simulink model "fullWaveUncontrolledRectifier_Rload"  (R2024b)
settings: Solver=ode23t  StartTime=0.0  StopTime=0.16  MaxStep=1e-4  RelTol=1e-3
libraries: spsDiodeLib x4, spsSeriesRLCBranchLib x3, spsVoltageMeasurementLib x2, spsACVoltageSourceLib x1, spsLinearTransformerLib x1, spsCurrentMeasurementLib x1, sps_lib x1
settings Model: Creator=farha  LastModifiedBy=farha

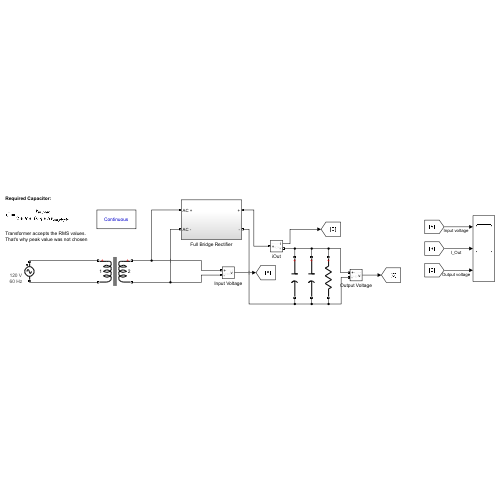
[thumbnail: Simulink's stored preview of the top-level diagram]
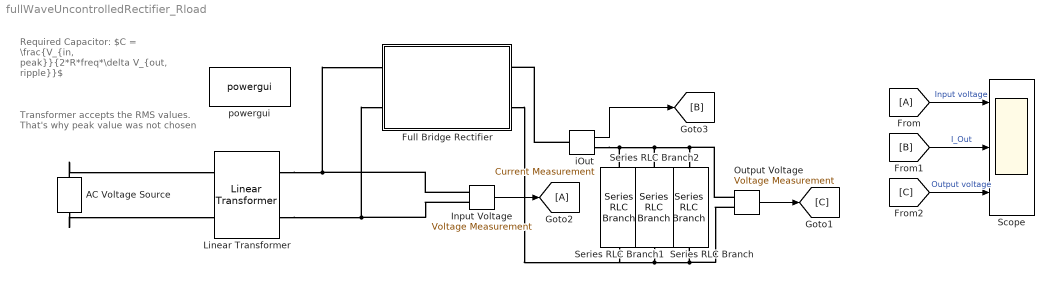
== system fullWaveUncontrolledRectifier_Rload ==
  note: Transformer accepts the RMS values.
      | That's why peak value was not chosen
  note: Required Capacitor:
      |
      | $C = \frac{V_{in, peak}}{2*R*freq*\delta V_{out, ripple}}$
  AC Voltage Source : spsACVoltageSourceLib/AC Voltage Source  Amplitude=120  Phase=0  Frequency=60  SampleTime=0  Measurements=None  BusType=swing  Pref=10e3  Qref=0  Qmin=-inf  Qmax=+inf
      settings: AttributesFormatString=|
      | %<Amplitude> V
      | %<Frequency> Hz
  From : From
  Full Bridge Rectifier : Subsystem
  Goto2 : Goto
  Input Voltage : spsVoltageMeasurementLib/Voltage Measurement  PhasorSimulation=off  OutputType=Complex  PSBequivalent=0
  Linear Transformer : spsLinearTransformerLib/Linear Transformer  UNITS=pu  NominalPower=[ 300 60 ]  winding1=[ 120 0 0 ]  winding2="[ 25.6  0  0 ]"  ThreeWindings=off  winding3=[ 315e3 0.002 0.08 ]  RmLm=[ 500 500 ]  Measurements=None  DataType=off
  Output Voltage : spsVoltageMeasurementLib/Voltage Measurement  PhasorSimulation=off  OutputType=Complex  PSBequivalent=0
  Scope : Scope  NumInputPorts=3
  Series RLC Branch : spsSeriesRLCBranchLib/Series RLC Branch  LConnTagsString=__new0  RConnTagsString=__new0  BranchType=R  Resistance=500  Inductance=1e-3  SetiL0=off  InitialCurrent=0  Capacitance=1e-6  Setx0=off  InitialVoltage=0  Measurements=None
  Series RLC Branch1 : spsSeriesRLCBranchLib/Series RLC Branch  LConnTagsString=__new0  RConnTagsString=__new0  BranchType=C  Resistance=5  Inductance=1e-3  SetiL0=off  InitialCurrent=0  Capacitance=47e-6  Setx0=off  InitialVoltage=0  Measurements=None
  Series RLC Branch2 : spsSeriesRLCBranchLib/Series RLC Branch  LConnTagsString=__new0  RConnTagsString=__new0  BranchType=C  Resistance=5  Inductance=1e-3  SetiL0=off  InitialCurrent=0  Capacitance=47e-6  Setx0=off  InitialVoltage=0  Measurements=None
  iOut : spsCurrentMeasurementLib/Current Measurement  PhasorSimulation=off  OutputType=Complex  PSBequivalent=0
  powergui : sps_lib/powergui  Priority=1  SimulationMode=Continuous  SampleTime=50e-6  frequency=60  Iterations=50  frequencyindice=60  Pbase=100e6  ErrMax=1e-4  UnitsV=kV  UnitsW=MW  buscounter=0  FunctionMessages=off  echomessages=off  EnableUseOfTLC=off  CurrentSourceSwitches=off  DisableSnubberDevices=off  DisableRonSwitches=off  DisableVfSwitches=off  DisplayEquations=off  AutomaticDiscreteSolvers=off  SolverType=Tustin/Backward Euler (TBE)  Interpol=off  ExternalGateDelay=off  methode=off  Ts=100  x0status=blocks  SPID=on  SwTol=0  HookPort=off  NonlinearTolerance=1e-4  nMaxIteration=100  ContinueOnMaxIteration=off  RestoreLinks=warning  ResistiveCurrentMeasurement=off  Frange=[0:2:500]  Ylog=off  Xlog=on  ShowGrid=off  save=off  variable=ZData  structure=0  ZoomFFT=off  StartTime=0.0  cycles=1  DisplayStyle=1  fundamental=60  FreqAxis=off  MaxFrequency=1000  frequencyindicesteady=1  RmsSteady=1  display=off
  wires:
  From/1 -> Scope/1  "Input voltage"
  [B] -> Scope/2  "I_Out"
  [C] -> Scope/3  "Output voltage"
  Output Voltage/1 -> [C]
  iOut/1 -> [B]
  Input Voltage/1 -> Goto2/1
  connections:
  iOut/RConn1 -- Series RLC Branch2/LConn1 -- Output Voltage/LConn1 -- Series RLC Branch/LConn1 -- Series RLC Branch1/LConn1
  Input Voltage/LConn1 -- Full Bridge Rectifier/LConn1 -- Linear Transformer/RConn1
  Input Voltage/LConn2 -- Linear Transformer/RConn2 -- Full Bridge Rectifier/LConn2
  Output Voltage/LConn2 -- Series RLC Branch2/RConn1 -- Series RLC Branch1/RConn1 -- Full Bridge Rectifier/RConn2 -- Series RLC Branch/RConn1
  iOut/LConn1 -- Full Bridge Rectifier/RConn1
  AC Voltage Source/RConn1 -- Linear Transformer/LConn1
  AC Voltage Source/LConn1 -- Linear Transformer/LConn2

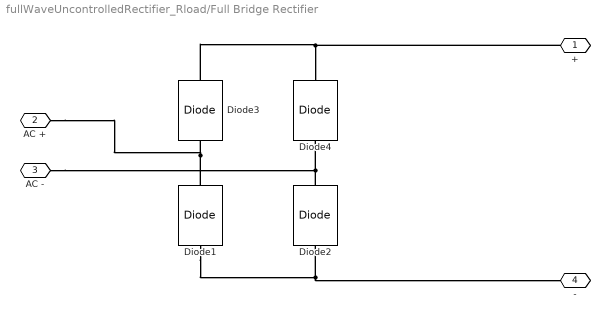
== system fullWaveUncontrolledRectifier_Rload/Full Bridge Rectifier ==
  Diode{1..4} (4 alike) : spsDiodeLib/Diode  Ron=0.001  Lon=0  Vf=0.6  IC=0  UseSnubber=0  Rs=500  Cs=250e-9  Measurements=off
  + : PMIOPort  Side=Right
  AC + : PMIOPort  Port=2  Side=Left
  AC - : PMIOPort  Port=3  Side=Left
  - : PMIOPort  Port=4  Side=Right
  connections:
  Diode1/RConn1 -- AC +/RConn1 -- Diode3/LConn1
  Diode3/RConn1 -- +/RConn1 -- Diode4/RConn1
  Diode2/RConn1 -- Diode4/LConn1 -- AC -/RConn1
  Diode1/LConn1 -- -/RConn1 -- Diode2/LConn1
